simulink model "ntc_measure"  (R2024a)
settings: Solver=ode1be  StartTime=0.0  StopTime=simlength  FixedStep=tc  RelTol=1e-3
undefined symbols (not defined in the file or in its folder): open_loop_gain_opa350, Rntc, tc
libraries: fl_lib x177, ee_lib x28, nesl_utility x26
(part 2 of 2)

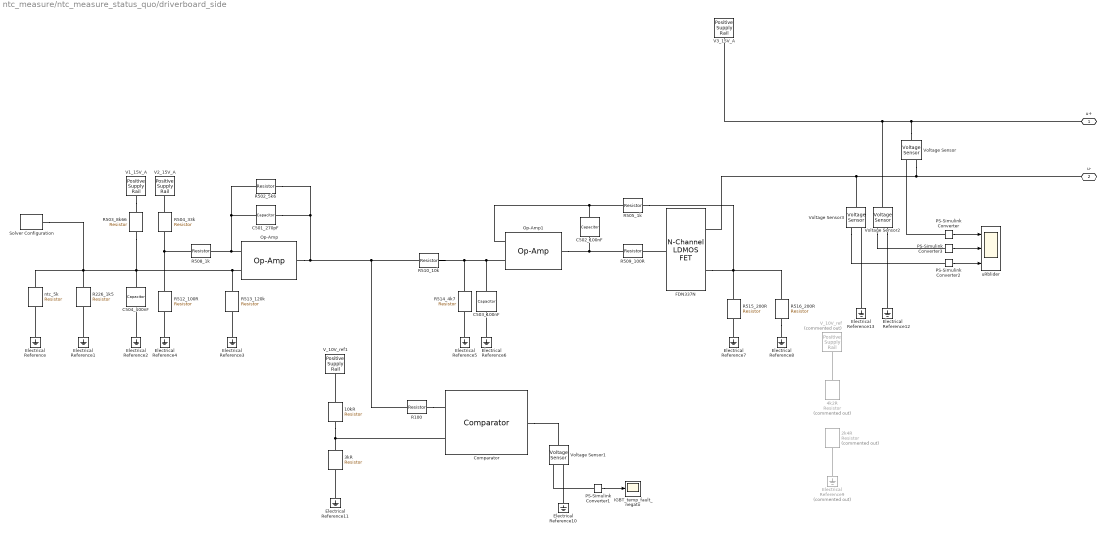
== system ntc_measure/ntc_measure_status_quo/driverboard_side ==
  10kR : fl_lib/Electrical/Electrical Elements/Resistor  R=10e3 Ohm  i_specify=off  i_priority=None  i=0 A  i_nominal_specify=off  i_nominal_value=1  i_nominal_unit=A  v_specify=off  v_priority=None  v=0 V  v_nominal_specify=off  v_nominal_value=1  v_nominal_unit=V
  2k4R : fl_lib/Electrical/Electrical Elements/Resistor  Commented=on  R=2.4e3 Ohm  i_specify=off  i_priority=None  i=0 A  i_nominal_specify=off  i_nominal_value=1  i_nominal_unit=A  v_specify=off  v_priority=None  v=0 V  v_nominal_specify=off  v_nominal_value=1  v_nominal_unit=V
  3kR : fl_lib/Electrical/Electrical Elements/Resistor  R=3e3 Ohm  i_specify=off  i_priority=None  i=0 A  i_nominal_specify=off  i_nominal_value=1  i_nominal_unit=A  v_specify=off  v_priority=None  v=0 V  v_nominal_specify=off  v_nominal_value=1  v_nominal_unit=V
  4k2R : fl_lib/Electrical/Electrical Elements/Resistor  Commented=on  R=4.2e3 Ohm  i_specify=off  i_priority=None  i=0 A  i_nominal_specify=off  i_nominal_value=1  i_nominal_unit=A  v_specify=off  v_priority=None  v=0 V  v_nominal_specify=off  v_nominal_value=1  v_nominal_unit=V
  C501_270pF : fl_lib/Electrical/Electrical Elements/Capacitor  c=270e-12 F  r=1e-6 Ohm  g=0 1/Ohm  i_specify=off  i_priority=None  i=0 A  i_nominal_specify=off  i_nominal_value=1  i_nominal_unit=A  v_specify=off  v_priority=None  v=0 V  v_nominal_specify=off  v_nominal_value=1  v_nominal_unit=V  vc_specify=off  vc_priority=High  vc=0 V  vc_nominal_specify=off  vc_nominal_value=1  vc_nominal_unit=V
  C502_100nF : fl_lib/Electrical/Electrical Elements/Capacitor  c=100e-9 F  r=1e-6 Ohm  g=0 1/Ohm  i_specify=off  i_priority=None  i=0 A  i_nominal_specify=off  i_nominal_value=1  i_nominal_unit=A  v_specify=off  v_priority=None  v=0 V  v_nominal_specify=off  v_nominal_value=1  v_nominal_unit=V  vc_specify=off  vc_priority=High  vc=0 V  vc_nominal_specify=off  vc_nominal_value=1  vc_nominal_unit=V
  C503_100nF : fl_lib/Electrical/Electrical Elements/Capacitor  c=100e-9 F  r=1e-6 Ohm  g=0 1/Ohm  i_specify=off  i_priority=None  i=0 A  i_nominal_specify=off  i_nominal_value=1  i_nominal_unit=A  v_specify=off  v_priority=None  v=0 V  v_nominal_specify=off  v_nominal_value=1  v_nominal_unit=V  vc_specify=off  vc_priority=High  vc=0 V  vc_nominal_specify=off  vc_nominal_value=1  vc_nominal_unit=V
  C504_100nF : fl_lib/Electrical/Electrical Elements/Capacitor  c=100e-9 F  r=1e-6 Ohm  g=0 1/Ohm  i_specify=off  i_priority=None  i=0 A  i_nominal_specify=off  i_nominal_value=1  i_nominal_unit=A  v_specify=off  v_priority=None  v=0 V  v_nominal_specify=off  v_nominal_value=1  v_nominal_unit=V  vc_specify=off  vc_priority=High  vc=0 V  vc_nominal_specify=off  vc_nominal_value=1  vc_nominal_unit=V
  Comparator : ee_lib/Integrated Circuits/Comparator  V_OS=5 mV  C_IN=0 pF  V_OL=0 V  V_OH=5 V  R_OUT=50 Ohm  Delay=0 s
      settings: InternalSimscapePortConfiguration="{\"Bottom\":[],\"Left\":[{\"id\":\"p\",\"label\":\"+\",\"type\":\"foundation.electrical.electrical\"},{\"id\":\"n\",\"label\":\"-\",\"type\":\"foundation.electrical.electrical\"}],\"Right\":[{\"id\":\"J\",\"label\":\"\",\"type\":\"foundation.electrical.electrical\"}],\"Top\":[]}"
  Electrical Reference{,1..8,10..13} (13 alike) : fl_lib/Electrical/Electrical Elements/Electrical Reference
  Electrical Reference9 : fl_lib/Electrical/Electrical Elements/Electrical Reference  Commented=on
  FDN337N : ee_lib/Semiconductors & Converters/N-Channel LDMOS FET  betaref=[11.6, .01] A/V^2  Vfbref=[-1.05, -.1] V  gamma=[3.4, 2.5] V^(1/2)  phib2ref=[.95, .95] V  thesatref=[0, .1] 1/V  theaccdr=0 1/V  alpha=0  Vp=5e-2 V  m=8  Tmeas=25 degC  Rsref=1e-4 Ohm  Rdref=0.07 Ohm  Rgref=8.4 Ohm  Rdriftref=0.1 Ohm  lambda=0.2  Cox=[1600, 1000] pF  Cgso=15 pF  Cgdo=15 pF  Isref=1e-13 A  Vbi=0.6 V  n=1  Cj0=1800 pF  TT=50e-9 s  Tprm=1  Tsim=25 degC  etabet=[1.3, 1.3]  Stvfb=[.0005, .0005] V/K  Stphib=-8.5e-4 V/K  etasat=[1.04, 1.04]  etar=0.95  etardr=0.95  etais=3  Ig_specify=off  Ig_priority=None  Ig=0 A  Ig_nominal_specify=off  Ig_nominal_value=1  Ig_nominal_unit=A  Id_specify=off  Id_priority=None  Id=0 A  Id_nominal_specify=off  Id_nominal_value=1  Id_nominal_unit=A  V_gs_specify=off  V_gs_priority=None  V_gs=0 V  V_gs_nominal_specify=off  V_gs_nominal_value=1  V_gs_nominal_unit=V  V_ds_specify=off  V_ds_priority=None  V_ds=0 V  V_ds_nominal_specify=off  V_ds_nominal_value=1  V_ds_nominal_unit=V  QGoverCox_specify=off  QGoverCox_priority=Low  QGoverCox=0 V  QGoverCox_nominal_specify=off  QGoverCox_nominal_value=1  QGoverCox_nominal_unit=V  QDoverCox_specify=off  QDoverCox_priority=Low  QDoverCox=0 V  QDoverCox_nominal_specify=off  QDoverCox_nominal_value=1  QDoverCox_nominal_unit=V  thermal_network_parameterization=ee.enum.thermalNetworkTopology.junctionCase  Rth=[0, 10] K/W  Rth_Cauer=[1, 3, 10] K/W  Rth_Foster=[4, 6] K/W  thermal_mass_parameterization=ee.enum.thermalNetwork.timeconstant  thermal_mass=[0, 1] J/K  thermal_mass_Cauer=[.1, .3, 1] J/K  thermal_mass_Foster=[1.5, 3] J/K  thermal_time_constant=[0, 10] s  thermal_time_constant_Cauer=[1, 3, 10] s  thermal_time_constant_Foster=[6, 18] s  T0=[25, 25] degC  T0_Cauer=[25, 25, 25] degC  Tvec_initial_Foster=[25, 25, 25, 25] degC
      settings: InternalSimscapePortConfiguration="{\"Bottom\":[],\"Left\":[{\"id\":\"G\",\"label\":\"\",\"type\":\"foundation.electrical.electrical\"}],\"Right\":[{\"id\":\"D\",\"label\":\"d\",\"type\":\"foundation.electrical.electrical\"},{\"id\":\"S\",\"label\":\"s\",\"type\":\"foundation.electrical.electrical\"}],\"Top\":[]}"
  IGBT_temp_fault_negato : Scope
  Op-Amp : fl_lib/Electrical/Electrical Elements/Op-Amp  outI_specify=off  outI_priority=None  outI=0 A  outI_nominal_specify=off  outI_nominal_value=1  outI_nominal_unit=A
  Op-Amp1 : fl_lib/Electrical/Electrical Elements/Op-Amp  outI_specify=off  outI_priority=None  outI=0 A  outI_nominal_specify=off  outI_nominal_value=1  outI_nominal_unit=A
  PS-Simulink Converter{,1..3} (4 alike) : nesl_utility/PS-Simulink Converter  PhysicalDomain=network_engine_domain  SubClassName=ps_output  LeftPortType=input  RightPortType=output  PseudoPeriodic=off  Frequencies=[]  VectorFormat=1-D array  Unit=V  AffineConversion=off
  R100 : fl_lib/Electrical/Electrical Elements/Resistor  R=100 Ohm  i_specify=off  i_priority=None  i=0 A  i_nominal_specify=off  i_nominal_value=1  i_nominal_unit=A  v_specify=off  v_priority=None  v=0 V  v_nominal_specify=off  v_nominal_value=1  v_nominal_unit=V
  R226_1k5 : fl_lib/Electrical/Electrical Elements/Resistor  R=1.5e3 Ohm  i_specify=off  i_priority=None  i=0 A  i_nominal_specify=off  i_nominal_value=1  i_nominal_unit=A  v_specify=off  v_priority=None  v=0 V  v_nominal_specify=off  v_nominal_value=1  v_nominal_unit=V
  R502_5k6 : fl_lib/Electrical/Electrical Elements/Resistor  R=5.6e3 Ohm  i_specify=off  i_priority=None  i=0 A  i_nominal_specify=off  i_nominal_value=1  i_nominal_unit=A  v_specify=off  v_priority=None  v=0 V  v_nominal_specify=off  v_nominal_value=1  v_nominal_unit=V
  R503_8k66 : fl_lib/Electrical/Electrical Elements/Resistor  R=8.66e3 Ohm  i_specify=off  i_priority=None  i=0 A  i_nominal_specify=off  i_nominal_value=1  i_nominal_unit=A  v_specify=off  v_priority=None  v=0 V  v_nominal_specify=off  v_nominal_value=1  v_nominal_unit=V
  R504_33k : fl_lib/Electrical/Electrical Elements/Resistor  R=33e3 Ohm  i_specify=off  i_priority=None  i=0 A  i_nominal_specify=off  i_nominal_value=1  i_nominal_unit=A  v_specify=off  v_priority=None  v=0 V  v_nominal_specify=off  v_nominal_value=1  v_nominal_unit=V
  R505_1k : fl_lib/Electrical/Electrical Elements/Resistor  R=1e3 Ohm  i_specify=off  i_priority=None  i=0 A  i_nominal_specify=off  i_nominal_value=1  i_nominal_unit=A  v_specify=off  v_priority=None  v=0 V  v_nominal_specify=off  v_nominal_value=1  v_nominal_unit=V
  R508_1k : fl_lib/Electrical/Electrical Elements/Resistor  R=1e3 Ohm  i_specify=off  i_priority=None  i=0 A  i_nominal_specify=off  i_nominal_value=1  i_nominal_unit=A  v_specify=off  v_priority=None  v=0 V  v_nominal_specify=off  v_nominal_value=1  v_nominal_unit=V
  R509_100R : fl_lib/Electrical/Electrical Elements/Resistor  R=100 Ohm  i_specify=off  i_priority=None  i=0 A  i_nominal_specify=off  i_nominal_value=1  i_nominal_unit=A  v_specify=off  v_priority=None  v=0 V  v_nominal_specify=off  v_nominal_value=1  v_nominal_unit=V
  R510_10k : fl_lib/Electrical/Electrical Elements/Resistor  R=10e3 Ohm  i_specify=off  i_priority=None  i=0 A  i_nominal_specify=off  i_nominal_value=1  i_nominal_unit=A  v_specify=off  v_priority=None  v=0 V  v_nominal_specify=off  v_nominal_value=1  v_nominal_unit=V
  R512_100R : fl_lib/Electrical/Electrical Elements/Resistor  R=100 Ohm  i_specify=off  i_priority=None  i=0 A  i_nominal_specify=off  i_nominal_value=1  i_nominal_unit=A  v_specify=off  v_priority=None  v=0 V  v_nominal_specify=off  v_nominal_value=1  v_nominal_unit=V
  R513_120k : fl_lib/Electrical/Electrical Elements/Resistor  R=120e3 Ohm  i_specify=off  i_priority=None  i=0 A  i_nominal_specify=off  i_nominal_value=1  i_nominal_unit=A  v_specify=off  v_priority=None  v=0 V  v_nominal_specify=off  v_nominal_value=1  v_nominal_unit=V
  R514_4k7 : fl_lib/Electrical/Electrical Elements/Resistor  R=4.7e3 Ohm  i_specify=off  i_priority=None  i=0 A  i_nominal_specify=off  i_nominal_value=1  i_nominal_unit=A  v_specify=off  v_priority=None  v=0 V  v_nominal_specify=off  v_nominal_value=1  v_nominal_unit=V
  R515_200R : fl_lib/Electrical/Electrical Elements/Resistor  R=200 Ohm  i_specify=off  i_priority=None  i=0 A  i_nominal_specify=off  i_nominal_value=1  i_nominal_unit=A  v_specify=off  v_priority=None  v=0 V  v_nominal_specify=off  v_nominal_value=1  v_nominal_unit=V
  R516_200R : fl_lib/Electrical/Electrical Elements/Resistor  R=200 Ohm  i_specify=off  i_priority=None  i=0 A  i_nominal_specify=off  i_nominal_value=1  i_nominal_unit=A  v_specify=off  v_priority=None  v=0 V  v_nominal_specify=off  v_nominal_value=1  v_nominal_unit=V
  Solver Configuration : nesl_utility/Solver Configuration  PhysicalDomain=network_engine_domain  SubClassName=solver  LeftPortType=input  RightPortType=generic  Tones=[]  Harmonics=[]  SimulateNoise=off  Profile=off  UseLocalSampling=off  EnableSwitchedLinearOptims=on  FrequencyDomain=off  UseCCode=off  RelTol=0.001  AbsTol=0.001  MinStep=1e-09  ToWorkspace=off  RevertToSquareIcSolve=off  NumHomotopyIterations=100  PhasorMode=off  PhasorModeNumHarmonics=1  ConsistencySolver=NEWTON_XTOL_AFTER_FTOL  IndexReductionMethod=DerivativeReplacement  DoDC=off  ResidualTolerance=1e-09  ConsistencyTolSource=GLOBAL  ConsistencyAbsTol=0.001  ConsistencyRelTol=0.001  ConsistencyTolFactor=0.001  UseLocalSolver=on  LocalSolverChoice=NE_BACKWARD_EULER_ADVANCER  ResolveIndetEquations=on  FunctionEvalNumThread=1  LocalSolverSampleTime=tc  DoFixedCost=on  MaxNonlinIter=3  MaxModeIter=2  ComputeImpulses=off  ImpulseIterations=2  LinearAlgebra=auto  LinearAlgebraNumThread=0  EquationFormulation=NE_TIME_EF  DelaysMemoryBudget=1024  AutomaticFiltering=on  FilteringTimeConstant=0.001  PartitionStorageMethod=AS_NEEDED  PartitionMemoryBudget=1024  PartitionMethod=ROBUST  MultibodyUseLocalSolver=off  MultibodyLocalSolverChoice=ODE1  MultibodyLocalSolverSampleTime=0.001
  V1_15V_A : ee_lib/Sources/Positive Supply Rail  v0=15 V
      settings: InternalSimscapePortConfiguration="{\"Bottom\":[],\"Left\":[],\"Right\":[{\"id\":\"p\",\"label\":\"\",\"type\":\"foundation.electrical.electrical\"}],\"Top\":[]}"
  V2_15V_A : ee_lib/Sources/Positive Supply Rail  v0=15 V
      settings: InternalSimscapePortConfiguration="{\"Bottom\":[],\"Left\":[],\"Right\":[{\"id\":\"p\",\"label\":\"\",\"type\":\"foundation.electrical.electrical\"}],\"Top\":[]}"
  V3_15V_A : ee_lib/Sources/Positive Supply Rail  v0=15 V
      settings: InternalSimscapePortConfiguration="{\"Bottom\":[],\"Left\":[],\"Right\":[{\"id\":\"p\",\"label\":\"\",\"type\":\"foundation.electrical.electrical\"}],\"Top\":[]}"
  V_10V_ref : ee_lib/Sources/Positive Supply Rail  Commented=on  v0=10 V
      settings: InternalSimscapePortConfiguration="{\"Bottom\":[],\"Left\":[],\"Right\":[{\"id\":\"p\",\"label\":\"\",\"type\":\"foundation.electrical.electrical\"}],\"Top\":[]}"
  V_10V_ref1 : ee_lib/Sources/Positive Supply Rail  v0=10 V
      settings: InternalSimscapePortConfiguration="{\"Bottom\":[],\"Left\":[],\"Right\":[{\"id\":\"p\",\"label\":\"\",\"type\":\"foundation.electrical.electrical\"}],\"Top\":[]}"
  Voltage Sensor{,1..3} (4 alike) : fl_lib/Electrical/Electrical Sensors/Voltage Sensor
  ntc_5k : fl_lib/Electrical/Electrical Elements/Resistor  R=Rntc Ohm  i_specify=off  i_priority=None  i=0 A  i_nominal_specify=off  i_nominal_value=1  i_nominal_unit=A  v_specify=off  v_priority=None  v=0 V  v_nominal_specify=off  v_nominal_value=1  v_nominal_unit=V
  uRblider : Scope  NumInputPorts=3
  u+ : PMIOPort  Side=Right
  u- : PMIOPort  Port=2  Side=Right
  wires:
  PS-Simulink Converter/1 -> uRblider/1
  PS-Simulink Converter1/1 -> IGBT_temp_fault_negato/1
  PS-Simulink Converter2/1 -> uRblider/3
  PS-Simulink Converter3/1 -> uRblider/2
  connections:
  Electrical Reference7/LConn1 -- R515_200R/RConn1
  Voltage Sensor/LConn1 -- u+/RConn1 -- Voltage Sensor2/LConn1 -- V3_15V_A/RConn1
  R508_1k/LConn1 -- R512_100R/LConn1 -- R504_33k/RConn1
  R503_8k66/RConn1 -- R226_1k5/LConn1 -- Solver Configuration/RConn1 -- ntc_5k/LConn1 -- Op-Amp/LConn1 -- R513_120k/LConn1 -- C504_100nF/LConn1
  Electrical Reference5/LConn1 -- R514_4k7/RConn1
  Voltage Sensor/RConn2 -- u-/RConn1 -- Voltage Sensor3/LConn1 -- FDN337N/RConn1
  R504_33k/LConn1 -- V2_15V_A/RConn1
  Op-Amp1/LConn2 -- C502_100nF/LConn1 -- R505_1k/LConn1
  R508_1k/RConn1 -- Op-Amp/LConn2 -- R502_5k6/LConn1 -- C501_270pF/LConn1
  FDN337N/LConn1 -- R509_100R/RConn1
  FDN337N/RConn2 -- R505_1k/RConn1 -- R515_200R/LConn1 -- R516_200R/LConn1
  Op-Amp1/RConn1 -- C502_100nF/RConn1 -- R509_100R/LConn1
  Electrical Reference/LConn1 -- ntc_5k/RConn1
  V1_15V_A/RConn1 -- R503_8k66/LConn1
  Electrical Reference1/LConn1 -- R226_1k5/RConn1
  Electrical Reference2/LConn1 -- C504_100nF/RConn1
  R510_10k/RConn1 -- C503_100nF/LConn1 -- Op-Amp1/LConn1 -- R514_4k7/LConn1
  C501_270pF/RConn1 -- R100/LConn1 -- R510_10k/LConn1 -- Op-Amp/RConn1 -- R502_5k6/RConn1
  Electrical Reference6/LConn1 -- C503_100nF/RConn1
  Electrical Reference3/LConn1 -- R513_120k/RConn1
  Electrical Reference4/LConn1 -- R512_100R/RConn1
  PS-Simulink Converter/LConn1 -- Voltage Sensor/RConn1
  R516_200R/RConn1 -- Electrical Reference8/LConn1
  4k2R/LConn1 -- V_10V_ref/RConn1
  Electrical Reference9/LConn1 -- 2k4R/RConn1
  R100/RConn1 -- Comparator/LConn1
  Comparator/RConn1 -- Voltage Sensor1/LConn1
  PS-Simulink Converter1/LConn1 -- Voltage Sensor1/RConn1
  Electrical Reference10/LConn1 -- Voltage Sensor1/RConn2
  10kR/RConn1 -- Comparator/LConn2 -- 3kR/LConn1
  Electrical Reference11/LConn1 -- 3kR/RConn1
  10kR/LConn1 -- V_10V_ref1/RConn1
  Voltage Sensor2/RConn2 -- Electrical Reference12/LConn1
  Electrical Reference13/LConn1 -- Voltage Sensor3/RConn2
  Voltage Sensor2/RConn1 -- PS-Simulink Converter3/LConn1
  Voltage Sensor3/RConn1 -- PS-Simulink Converter2/LConn1

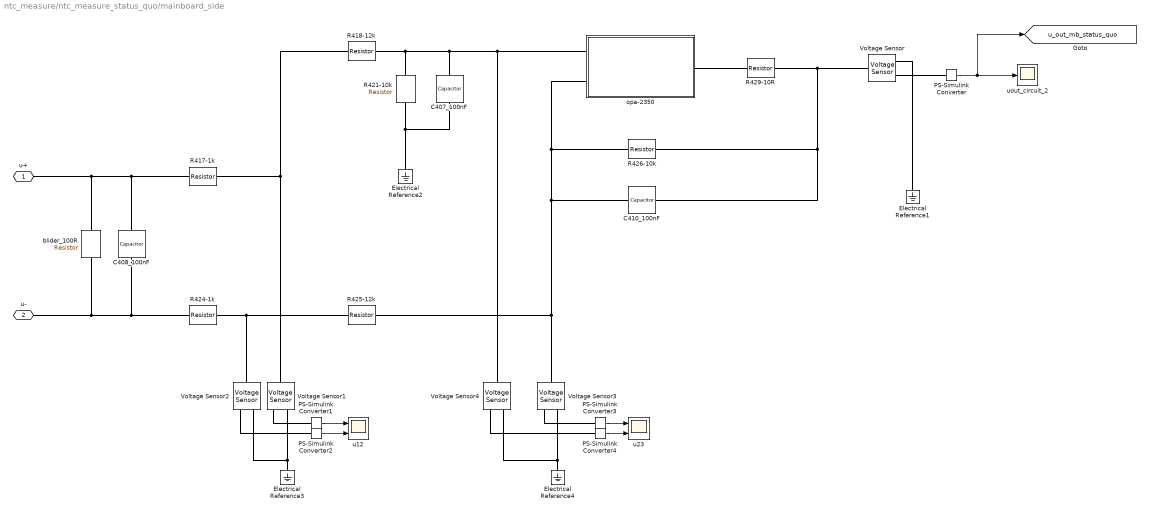
== system ntc_measure/ntc_measure_status_quo/mainboard_side ==
  C407_100nF : fl_lib/Electrical/Electrical Elements/Capacitor  c=100e-9 F  r=1e-6 Ohm  g=0 1/Ohm  i_specify=off  i_priority=None  i=0 A  i_nominal_specify=off  i_nominal_value=1  i_nominal_unit=A  v_specify=off  v_priority=None  v=0 V  v_nominal_specify=off  v_nominal_value=1  v_nominal_unit=V  vc_specify=off  vc_priority=High  vc=0 V  vc_nominal_specify=off  vc_nominal_value=1  vc_nominal_unit=V
  C408_100nF : fl_lib/Electrical/Electrical Elements/Capacitor  c=100e-9 F  r=1e-6 Ohm  g=0 1/Ohm  i_specify=off  i_priority=None  i=0 A  i_nominal_specify=off  i_nominal_value=1  i_nominal_unit=A  v_specify=off  v_priority=None  v=0 V  v_nominal_specify=off  v_nominal_value=1  v_nominal_unit=V  vc_specify=off  vc_priority=High  vc=0 V  vc_nominal_specify=off  vc_nominal_value=1  vc_nominal_unit=V
  C410_100nF : fl_lib/Electrical/Electrical Elements/Capacitor  c=100e-9 F  r=1e-6 Ohm  g=0 1/Ohm  i_specify=off  i_priority=None  i=0 A  i_nominal_specify=off  i_nominal_value=1  i_nominal_unit=A  v_specify=off  v_priority=None  v=0 V  v_nominal_specify=off  v_nominal_value=1  v_nominal_unit=V  vc_specify=off  vc_priority=High  vc=0 V  vc_nominal_specify=off  vc_nominal_value=1  vc_nominal_unit=V
  Electrical Reference{1..4} (4 alike) : fl_lib/Electrical/Electrical Elements/Electrical Reference
  PS-Simulink Converter{,1..4} (5 alike) : nesl_utility/PS-Simulink Converter  PhysicalDomain=network_engine_domain  SubClassName=ps_output  LeftPortType=input  RightPortType=output  PseudoPeriodic=off  Frequencies=[]  VectorFormat=1-D array  Unit=V  AffineConversion=off
  R417-1k : fl_lib/Electrical/Electrical Elements/Resistor  R=1e3 Ohm  i_specify=off  i_priority=None  i=0 A  i_nominal_specify=off  i_nominal_value=1  i_nominal_unit=A  v_specify=off  v_priority=None  v=0 V  v_nominal_specify=off  v_nominal_value=1  v_nominal_unit=V
  R418-12k : fl_lib/Electrical/Electrical Elements/Resistor  R=12e3 Ohm  i_specify=off  i_priority=None  i=0 A  i_nominal_specify=off  i_nominal_value=1  i_nominal_unit=A  v_specify=off  v_priority=None  v=0 V  v_nominal_specify=off  v_nominal_value=1  v_nominal_unit=V
  R421-10k : fl_lib/Electrical/Electrical Elements/Resistor  R=10e3 Ohm  i_specify=off  i_priority=None  i=0 A  i_nominal_specify=off  i_nominal_value=1  i_nominal_unit=A  v_specify=off  v_priority=None  v=0 V  v_nominal_specify=off  v_nominal_value=1  v_nominal_unit=V
  R424-1k : fl_lib/Electrical/Electrical Elements/Resistor  R=1e3 Ohm  i_specify=off  i_priority=None  i=0 A  i_nominal_specify=off  i_nominal_value=1  i_nominal_unit=A  v_specify=off  v_priority=None  v=0 V  v_nominal_specify=off  v_nominal_value=1  v_nominal_unit=V
  R425-12k : fl_lib/Electrical/Electrical Elements/Resistor  R=12e3 Ohm  i_specify=off  i_priority=None  i=0 A  i_nominal_specify=off  i_nominal_value=1  i_nominal_unit=A  v_specify=off  v_priority=None  v=0 V  v_nominal_specify=off  v_nominal_value=1  v_nominal_unit=V
  R426-10k : fl_lib/Electrical/Electrical Elements/Resistor  R=10e3 Ohm  i_specify=off  i_priority=None  i=0 A  i_nominal_specify=off  i_nominal_value=1  i_nominal_unit=A  v_specify=off  v_priority=None  v=0 V  v_nominal_specify=off  v_nominal_value=1  v_nominal_unit=V
  R429-10R : fl_lib/Electrical/Electrical Elements/Resistor  R=10 Ohm  i_specify=off  i_priority=None  i=0 A  i_nominal_specify=off  i_nominal_value=1  i_nominal_unit=A  v_specify=off  v_priority=None  v=0 V  v_nominal_specify=off  v_nominal_value=1  v_nominal_unit=V
  Voltage Sensor{,1..4} (5 alike) : fl_lib/Electrical/Electrical Sensors/Voltage Sensor
  blider_100R : fl_lib/Electrical/Electrical Elements/Resistor  R=100 Ohm  i_specify=off  i_priority=None  i=0 A  i_nominal_specify=off  i_nominal_value=1  i_nominal_unit=A  v_specify=off  v_priority=None  v=0 V  v_nominal_specify=off  v_nominal_value=1  v_nominal_unit=V
  opa-2350 : Subsystem  mask{V_opamp_pos=3.6, V_opamp_neg=-1.6, A=open_loop_gain_opa350}
      mask prompts: V_opamp_pos "V+"; V_opamp_neg "V-"; A "Open Loop Gain"
      mask help: rail to rail op-amp
      mask Help: eval('open opa2350.pdf')
      mask Display:
      | disp('OPA-2350');
      | port_label('lconn', 1, 'in(+)');
      | port_label('lconn', 2, 'in(-)');
      | port_label('rconn', 1, 'out');
  u12 : Scope  NumInputPorts=2
  u23 : Scope  NumInputPorts=2
  uout_circuit_2 : Scope
  u+ : PMIOPort  Side=Left
  u- : PMIOPort  Port=2  Side=Left
  tag scope: u_out_mb_status_quo=global
  wires:
  PS-Simulink Converter/1 -> [u_out_mb_status_quo], uout_circuit_2/1
  PS-Simulink Converter1/1 -> u12/1
  PS-Simulink Converter2/1 -> u12/2
  PS-Simulink Converter4/1 -> u23/2
  PS-Simulink Converter3/1 -> u23/1
  connections:
  R429-10R/LConn1 -- opa-2350/RConn1
  opa-2350/LConn2 -- C410_100nF/LConn1 -- R425-12k/LConn1 -- Voltage Sensor3/LConn1 -- R426-10k/LConn1
  u+/RConn1 -- blider_100R/LConn1 -- R417-1k/RConn1 -- C408_100nF/LConn1
  u-/RConn1 -- blider_100R/RConn1 -- R424-1k/RConn1 -- C408_100nF/RConn1
  Voltage Sensor1/LConn1 -- R417-1k/LConn1 -- R418-12k/RConn1
  Voltage Sensor2/LConn1 -- R424-1k/LConn1 -- R425-12k/RConn1
  opa-2350/LConn1 -- Voltage Sensor4/LConn1 -- C407_100nF/LConn1 -- R421-10k/LConn1 -- R418-12k/LConn1
  Electrical Reference2/LConn1 -- C407_100nF/RConn1 -- R421-10k/RConn1
  R429-10R/RConn1 -- C410_100nF/RConn1 -- R426-10k/RConn1 -- Voltage Sensor/LConn1
  Voltage Sensor/RConn2 -- Electrical Reference1/LConn1
  PS-Simulink Converter/LConn1 -- Voltage Sensor/RConn1
  Voltage Sensor1/RConn1 -- PS-Simulink Converter1/LConn1
  Voltage Sensor1/RConn2 -- Voltage Sensor2/RConn2 -- Electrical Reference3/LConn1
  Voltage Sensor2/RConn1 -- PS-Simulink Converter2/LConn1
  Voltage Sensor3/RConn2 -- Electrical Reference4/LConn1 -- Voltage Sensor4/RConn2
  Voltage Sensor4/RConn1 -- PS-Simulink Converter4/LConn1
  Voltage Sensor3/RConn1 -- PS-Simulink Converter3/LConn1

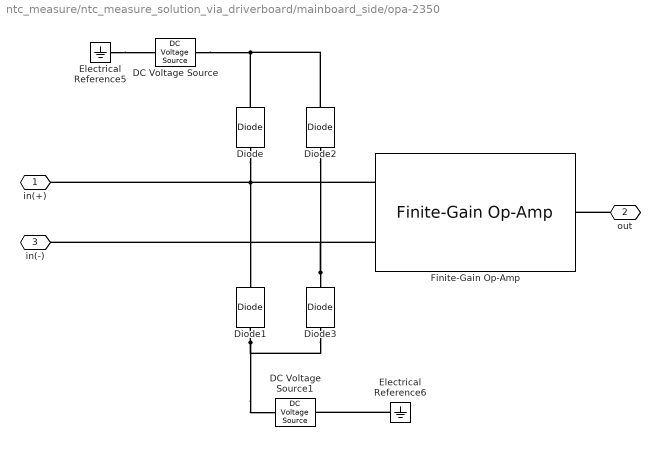
== system ntc_measure/ntc_measure_solution_via_driverboard/mainboard_side/opa-2350 ==
  DC Voltage Source : fl_lib/Electrical/Electrical Sources/DC Voltage Source  v0=V_opamp_pos V
  DC Voltage Source1 : fl_lib/Electrical/Electrical Sources/DC Voltage Source  v0=V_opamp_neg V
  Diode{,1..3} (4 alike) : ee_lib/Semiconductors & Converters/Diode  ModelType=ee.enum.diode.modelType.pwl  TableType=ee.enum.diode.tableType.IfMat  IfMat=[.07, .12, .19, 1.75, 4.24, 7.32, 11.2; .16, .3, .72, 2.14, 5.02, 8.35, 13.12] A  VfMat=[.9, 1.15, 1.25, 1.5, 1.75, 2.17, 2.6, 2.85; .58, .68, .75, 1.1, 1.38, 1.77, 2.27, 2.7] V  TjVec=[25, 125] degC  VfVec=[.5, .7, .9, 1.3, 1.7, 2.1, 2.5] V  IfVec=[.1, .2, .5, 1, 2, 4, 7, 10] A  IrMat=[1e-06, 2e-06, 5e-06, 1e-05, 2.5e-05, 5e-05, .0001; 2e-06, 5e-06, 1e-05, 4e-05, 8e-05, .0002, .0005] A  VrMat=[10, 100, 200, 250, 300, 325, 350; 10, 70, 160, 220, 270, 300, 320] V  VrVec=[10, 20, 40, 50, 70, 80, 100] V  IrVec=[1e-06, 2e-06, 5e-06, 1e-05, 2e-05, 5e-05, .0001] A  Vf=0.6 V  Ron=0.3 Ohm  Goff=1e-8 S  prmExp=ee.enum.diode.expParam.useTwo  I12=[.0137, .545] A  V12=[.6, .7] V  RS=0 Ohm  Tmeas=25 degC  IS=1e-12 A  ec=1  I1=0.0137 A  V1=0.6 V  N_series=1  N_parallel=1  ZenerEnable=false  Rz=0.3 Ohm  BV=inf V  C_param=ee.enum.diode.capParam.fixed  CJ=0 pF  CJ0=5 pF  Vvec=[.1, 10, 100] V  Cvec=[3.5, 1, .4] pF  VJ=1 V  Mgrad=0.5  FC=0.5  Q_param=ee.enum.diode.recoveryParam.off  iRM=-7.15 A  iF=4 A  didt=-750 A/us  trr_factor=3  trr=115 ns  Qrr=150 nA*s  Vr=-600 V  Ls=150 nH  Erec=0.03 J  TT=50 ns  tau=100 ns  T_param=ee.enum.diode.temperatureParam.off  Tdevice=25 degC  I1_T2=0.245 A  V1_T2=0.5 V  IS_T2=1.25e-7 A  Tmeas2=125 degC  XTI_param=ee.enum.diode.xtiParam.pn  XTI=3  EG_param=ee.enum.diode.egapParam.material_si  EG=1.11 eV  dBVdT=0 V/K  enable_faults=simscape.enum.onoff.off  fault_action=simscape.enum.assert.action.none  fault_types=ee.enum.diode.faults.open  tau_fault=1e-3 s  IfMat_faulted=[.07, .12, .19, 1.75, 4.24, 7.32, 11.2; .16, .3, .72, 2.14, 4.02, 6.35, 9.12] A  VfMat_faulted=[.9, 1.15, 1.25, 1.5, 1.75, 2.17, 2.6, 2.85; .58, .68, .75, 1.1, 1.38, 1.77, 2.27, 2.7] V  VfVec_faulted=[.5, .7, .9, 1.3, 1.7, 2.1, 2.5] V  IfVec_faulted=[.1, .2, .5, 1, 2, 4, 7, 10] A  IrMat_faulted=[1e-06, 2e-06, 5e-06, 1e-05, 2.5e-05, 5e-05, .0001; 2e-06, 5e-06, 1e-05, 4e-05, 8e-05, .0002, .0005] A  VrMat_faulted=[1, 10, 20, 25, 30, 32.5, 35; 1, 5, 10, 20, 25, 30, 32] V  VrVec_faulted=[1, 2, 4, 5, 7, 8, 10] V  IrVec_faulted=[1e-06, 2e-06, 5e-06, 1e-05, 2e-05, 5e-05, .0001] A  Ropen_faulted=1000 Ohm  Gshort_faulted=1000 1/Ohm  Vf_faulted=0.6 V  Ron_faulted=0.3 Ohm  Goff_faulted=1e-8 S  I12_faulted=[.0137, .545] A  V12_faulted=[.6, .7] V  IS_faulted=1e-12 A  ec_faulted=1  I1_faulted=0.0137 A  V1_faulted=0.6 V  RS_faulted=0 Ohm  Rz_faulted=0.3 Ohm  BV_faulted=inf V  Cscale_faulted=100  fault_trigger=ee.enum.faults.faultTrigger.temporal  t_fault=inf s  max_permissible_voltage=inf V  n_fail_on_voltage=1  max_permissible_current=inf A  t_fail_on_current=1 s  max_permissible_dVdt=inf V/s  enable_fault_input=simscape.enum.onoff.off  i_specify=off  i_priority=None  i=0 A  i_nominal_specify=off  i_nominal_value=1  i_nominal_unit=A  v_specify=off  v_priority=None  v=0 V  v_nominal_specify=off  v_nominal_value=1  v_nominal_unit=V  v_capacitor_specify=off  v_capacitor_priority=None  v_capacitor=0 V  v_capacitor_nominal_specify=off  v_capacitor_nominal_value=1  v_capacitor_nominal_unit=V  Qj_specify=off  Qj_priority=High  Qj=0 C  Qj_nominal_specify=off  Qj_nominal_value=1  Qj_nominal_unit=C  faulted_specify=off  faulted_priority=None  faulted=0  faulted_nominal_specify=off  faulted_nominal_value=1  faulted_nominal_unit=1  i_diode_specify=off  i_diode_priority=None  i_diode=0 A  i_diode_nominal_specify=off  i_diode_nominal_value=1  i_diode_nominal_unit=A  v_diode_specify=off  v_diode_priority=None  v_diode=0 V  v_diode_nominal_specify=off  v_diode_nominal_value=1  v_diode_nominal_unit=V  i_capacitor_specify=off  i_capacitor_priority=None  i_capacitor=0 A  i_capacitor_nominal_specify=off  i_capacitor_nominal_value=1  i_capacitor_nominal_unit=A  power_dissipated_specify=off  power_dissipated_priority=None  power_dissipated=0 W  power_dissipated_nominal_specify=off  power_dissipated_nominal_value=1  power_dissipated_nominal_unit=W  fidelity_level=ee.enum.diode.fidelity.includeChargeDyn  rec_loss_model=ee.enum.diode.reverseRecoveryModel.fixed  ErecVal=0 J  scaleWithIandV=true  ErecMat=zeros(2, 3) J  TjrecVec=[298.15, 398.15] K  IfrecVec=[.1, 1, 10] A  IrecVal=10 A  VrecVal=10 V  tFilter=1 / 1000 / 100 s  max_permissible_temperature=inf K  t_fail_on_temperature=1 s  thermal_network_parameterization=ee.enum.thermalNetworkTopology.junctionCase  Rth=[0, 10] K/W  Rth_Cauer=[1, 3, 10] K/W  Rth_Foster=[4, 6] K/W  thermal_mass_parameterization=ee.enum.thermalNetwork.timeconstant  thermal_mass=[0, 1] J/K  thermal_mass_Cauer=[.1, .3, 1] J/K  thermal_mass_Foster=[1.5, 3] J/K  thermal_time_constant=[0, 10] s  thermal_time_constant_Cauer=[1, 3, 10] s  thermal_time_constant_Foster=[6, 18] s  thermal_mass_initial_temperatures=[25, 25] degC  thermal_mass_initial_temperatures_Cauer=[25, 25, 25] degC  junction_thermal_mass=0.01 J/K  Tvec_initial_Foster=[25, 25, 25, 25] degC  no_thermal_network=0  junction_temperature_specify=off  junction_temperature_priority=None  junction_temperature=25 degC  junction_temperature_nominal_specify=off  junction_temperature_nominal_value=1  junction_temperature_nominal_unit=degC
  Electrical Reference5 : fl_lib/Electrical/Electrical Elements/Electrical Reference
  Electrical Reference6 : fl_lib/Electrical/Electrical Elements/Electrical Reference
  Finite-Gain Op-Amp : ee_lib/Integrated Circuits/Finite-Gain Op-Amp  A=A  Rin=1e6 Ohm  Rout=100 Ohm  Vmin=V_opamp_neg V  Vmax=V_opamp_pos V  noise_mode=ee.enum.mode.disabled  v_noise=30e-9 V/Hz^(1/2)  noise_prm=ee.enum.ic.noiseParameterization.same  i_noise=0.5e-12 A/Hz^(1/2)  ip_noise=0.5e-12 A/Hz^(1/2)  in_noise=0.5e-12 A/Hz^(1/2)  sample_time=1e-3 s  repeatability=ee.enum.ic.repeatability.notRepeatable  auto_seed_v=1196140742  auto_seed_ip=2348838240  auto_seed_in=4112460543  user_seed_v=0  user_seed_ip=0  user_seed_in=0
      settings: InternalSimscapePortConfiguration="{\"Bottom\":[],\"Left\":[{\"id\":\"p\",\"label\":\"+\",\"type\":\"foundation.electrical.electrical\"},{\"id\":\"n\",\"label\":\"-\",\"type\":\"foundation.electrical.electrical\"}],\"Right\":[{\"id\":\"out\",\"label\":\"\",\"type\":\"foundation.electrical.electrical\"}],\"Top\":[]}"
  in(+) : PMIOPort  Side=Left
  out : PMIOPort  Port=2  Side=Right
  in(-) : PMIOPort  Port=3  Side=Left
  connections:
  Finite-Gain Op-Amp/LConn1 -- in(+)/RConn1 -- Diode1/RConn1 -- Diode/LConn1
  Diode/RConn1 -- DC Voltage Source/LConn1 -- Diode2/RConn1
  out/RConn1 -- Finite-Gain Op-Amp/RConn1
  Diode3/RConn1 -- Diode2/LConn1 -- in(-)/RConn1 -- Finite-Gain Op-Amp/LConn2
  Diode1/LConn1 -- DC Voltage Source1/LConn1 -- Diode3/LConn1
  Electrical Reference6/LConn1 -- DC Voltage Source1/RConn1
  Electrical Reference5/LConn1 -- DC Voltage Source/RConn1

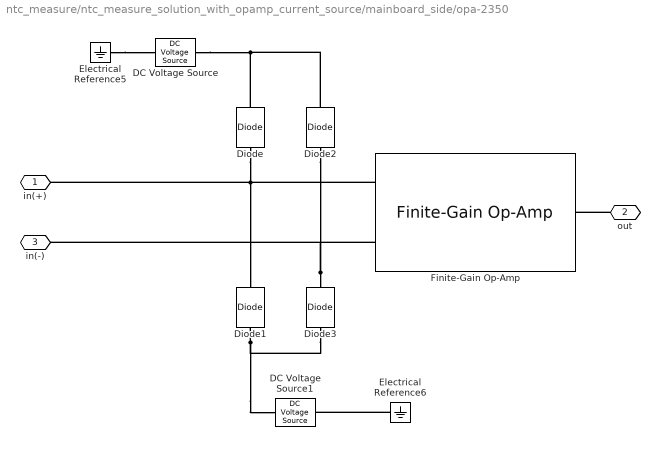
== system ntc_measure/ntc_measure_solution_with_opamp_current_source/mainboard_side/opa-2350 ==
  DC Voltage Source : fl_lib/Electrical/Electrical Sources/DC Voltage Source  v0=V_opamp_pos V
  DC Voltage Source1 : fl_lib/Electrical/Electrical Sources/DC Voltage Source  v0=V_opamp_neg V
  Diode{,1..3} (4 alike) : ee_lib/Semiconductors & Converters/Diode  ModelType=ee.enum.diode.modelType.pwl  TableType=ee.enum.diode.tableType.IfMat  IfMat=[.07, .12, .19, 1.75, 4.24, 7.32, 11.2; .16, .3, .72, 2.14, 5.02, 8.35, 13.12] A  VfMat=[.9, 1.15, 1.25, 1.5, 1.75, 2.17, 2.6, 2.85; .58, .68, .75, 1.1, 1.38, 1.77, 2.27, 2.7] V  TjVec=[25, 125] degC  VfVec=[.5, .7, .9, 1.3, 1.7, 2.1, 2.5] V  IfVec=[.1, .2, .5, 1, 2, 4, 7, 10] A  IrMat=[1e-06, 2e-06, 5e-06, 1e-05, 2.5e-05, 5e-05, .0001; 2e-06, 5e-06, 1e-05, 4e-05, 8e-05, .0002, .0005] A  VrMat=[10, 100, 200, 250, 300, 325, 350; 10, 70, 160, 220, 270, 300, 320] V  VrVec=[10, 20, 40, 50, 70, 80, 100] V  IrVec=[1e-06, 2e-06, 5e-06, 1e-05, 2e-05, 5e-05, .0001] A  Vf=0.6 V  Ron=0.3 Ohm  Goff=1e-8 S  prmExp=ee.enum.diode.expParam.useTwo  I12=[.0137, .545] A  V12=[.6, .7] V  RS=0 Ohm  Tmeas=25 degC  IS=1e-12 A  ec=1  I1=0.0137 A  V1=0.6 V  N_series=1  N_parallel=1  ZenerEnable=false  Rz=0.3 Ohm  BV=inf V  C_param=ee.enum.diode.capParam.fixed  CJ=0 pF  CJ0=5 pF  Vvec=[.1, 10, 100] V  Cvec=[3.5, 1, .4] pF  VJ=1 V  Mgrad=0.5  FC=0.5  Q_param=ee.enum.diode.recoveryParam.off  iRM=-7.15 A  iF=4 A  didt=-750 A/us  trr_factor=3  trr=115 ns  Qrr=150 nA*s  Vr=-600 V  Ls=150 nH  Erec=0.03 J  TT=50 ns  tau=100 ns  T_param=ee.enum.diode.temperatureParam.off  Tdevice=25 degC  I1_T2=0.245 A  V1_T2=0.5 V  IS_T2=1.25e-7 A  Tmeas2=125 degC  XTI_param=ee.enum.diode.xtiParam.pn  XTI=3  EG_param=ee.enum.diode.egapParam.material_si  EG=1.11 eV  dBVdT=0 V/K  enable_faults=simscape.enum.onoff.off  fault_action=simscape.enum.assert.action.none  fault_types=ee.enum.diode.faults.open  tau_fault=1e-3 s  IfMat_faulted=[.07, .12, .19, 1.75, 4.24, 7.32, 11.2; .16, .3, .72, 2.14, 4.02, 6.35, 9.12] A  VfMat_faulted=[.9, 1.15, 1.25, 1.5, 1.75, 2.17, 2.6, 2.85; .58, .68, .75, 1.1, 1.38, 1.77, 2.27, 2.7] V  VfVec_faulted=[.5, .7, .9, 1.3, 1.7, 2.1, 2.5] V  IfVec_faulted=[.1, .2, .5, 1, 2, 4, 7, 10] A  IrMat_faulted=[1e-06, 2e-06, 5e-06, 1e-05, 2.5e-05, 5e-05, .0001; 2e-06, 5e-06, 1e-05, 4e-05, 8e-05, .0002, .0005] A  VrMat_faulted=[1, 10, 20, 25, 30, 32.5, 35; 1, 5, 10, 20, 25, 30, 32] V  VrVec_faulted=[1, 2, 4, 5, 7, 8, 10] V  IrVec_faulted=[1e-06, 2e-06, 5e-06, 1e-05, 2e-05, 5e-05, .0001] A  Ropen_faulted=1000 Ohm  Gshort_faulted=1000 1/Ohm  Vf_faulted=0.6 V  Ron_faulted=0.3 Ohm  Goff_faulted=1e-8 S  I12_faulted=[.0137, .545] A  V12_faulted=[.6, .7] V  IS_faulted=1e-12 A  ec_faulted=1  I1_faulted=0.0137 A  V1_faulted=0.6 V  RS_faulted=0 Ohm  Rz_faulted=0.3 Ohm  BV_faulted=inf V  Cscale_faulted=100  fault_trigger=ee.enum.faults.faultTrigger.temporal  t_fault=inf s  max_permissible_voltage=inf V  n_fail_on_voltage=1  max_permissible_current=inf A  t_fail_on_current=1 s  max_permissible_dVdt=inf V/s  enable_fault_input=simscape.enum.onoff.off  i_specify=off  i_priority=None  i=0 A  i_nominal_specify=off  i_nominal_value=1  i_nominal_unit=A  v_specify=off  v_priority=None  v=0 V  v_nominal_specify=off  v_nominal_value=1  v_nominal_unit=V  v_capacitor_specify=off  v_capacitor_priority=None  v_capacitor=0 V  v_capacitor_nominal_specify=off  v_capacitor_nominal_value=1  v_capacitor_nominal_unit=V  Qj_specify=off  Qj_priority=High  Qj=0 C  Qj_nominal_specify=off  Qj_nominal_value=1  Qj_nominal_unit=C  faulted_specify=off  faulted_priority=None  faulted=0  faulted_nominal_specify=off  faulted_nominal_value=1  faulted_nominal_unit=1  i_diode_specify=off  i_diode_priority=None  i_diode=0 A  i_diode_nominal_specify=off  i_diode_nominal_value=1  i_diode_nominal_unit=A  v_diode_specify=off  v_diode_priority=None  v_diode=0 V  v_diode_nominal_specify=off  v_diode_nominal_value=1  v_diode_nominal_unit=V  i_capacitor_specify=off  i_capacitor_priority=None  i_capacitor=0 A  i_capacitor_nominal_specify=off  i_capacitor_nominal_value=1  i_capacitor_nominal_unit=A  power_dissipated_specify=off  power_dissipated_priority=None  power_dissipated=0 W  power_dissipated_nominal_specify=off  power_dissipated_nominal_value=1  power_dissipated_nominal_unit=W  fidelity_level=ee.enum.diode.fidelity.includeChargeDyn  rec_loss_model=ee.enum.diode.reverseRecoveryModel.fixed  ErecVal=0 J  scaleWithIandV=true  ErecMat=zeros(2, 3) J  TjrecVec=[298.15, 398.15] K  IfrecVec=[.1, 1, 10] A  IrecVal=10 A  VrecVal=10 V  tFilter=1 / 1000 / 100 s  max_permissible_temperature=inf K  t_fail_on_temperature=1 s  thermal_network_parameterization=ee.enum.thermalNetworkTopology.junctionCase  Rth=[0, 10] K/W  Rth_Cauer=[1, 3, 10] K/W  Rth_Foster=[4, 6] K/W  thermal_mass_parameterization=ee.enum.thermalNetwork.timeconstant  thermal_mass=[0, 1] J/K  thermal_mass_Cauer=[.1, .3, 1] J/K  thermal_mass_Foster=[1.5, 3] J/K  thermal_time_constant=[0, 10] s  thermal_time_constant_Cauer=[1, 3, 10] s  thermal_time_constant_Foster=[6, 18] s  thermal_mass_initial_temperatures=[25, 25] degC  thermal_mass_initial_temperatures_Cauer=[25, 25, 25] degC  junction_thermal_mass=0.01 J/K  Tvec_initial_Foster=[25, 25, 25, 25] degC  no_thermal_network=0  junction_temperature_specify=off  junction_temperature_priority=None  junction_temperature=25 degC  junction_temperature_nominal_specify=off  junction_temperature_nominal_value=1  junction_temperature_nominal_unit=degC
  Electrical Reference5 : fl_lib/Electrical/Electrical Elements/Electrical Reference
  Electrical Reference6 : fl_lib/Electrical/Electrical Elements/Electrical Reference
  Finite-Gain Op-Amp : ee_lib/Integrated Circuits/Finite-Gain Op-Amp  A=A  Rin=1e6 Ohm  Rout=100 Ohm  Vmin=V_opamp_neg V  Vmax=V_opamp_pos V  noise_mode=ee.enum.mode.disabled  v_noise=30e-9 V/Hz^(1/2)  noise_prm=ee.enum.ic.noiseParameterization.same  i_noise=0.5e-12 A/Hz^(1/2)  ip_noise=0.5e-12 A/Hz^(1/2)  in_noise=0.5e-12 A/Hz^(1/2)  sample_time=1e-3 s  repeatability=ee.enum.ic.repeatability.notRepeatable  auto_seed_v=3499211588  auto_seed_ip=3890346746  auto_seed_in=545404223  user_seed_v=0  user_seed_ip=0  user_seed_in=0
      settings: InternalSimscapePortConfiguration="{\"Bottom\":[],\"Left\":[{\"id\":\"p\",\"label\":\"+\",\"type\":\"foundation.electrical.electrical\"},{\"id\":\"n\",\"label\":\"-\",\"type\":\"foundation.electrical.electrical\"}],\"Right\":[{\"id\":\"out\",\"label\":\"\",\"type\":\"foundation.electrical.electrical\"}],\"Top\":[]}"
  in(+) : PMIOPort  Side=Left
  out : PMIOPort  Port=2  Side=Right
  in(-) : PMIOPort  Port=3  Side=Left
  connections:
  Finite-Gain Op-Amp/LConn1 -- in(+)/RConn1 -- Diode1/RConn1 -- Diode/LConn1
  Diode/RConn1 -- DC Voltage Source/LConn1 -- Diode2/RConn1
  out/RConn1 -- Finite-Gain Op-Amp/RConn1
  Diode3/RConn1 -- Diode2/LConn1 -- in(-)/RConn1 -- Finite-Gain Op-Amp/LConn2
  Diode1/LConn1 -- DC Voltage Source1/LConn1 -- Diode3/LConn1
  Electrical Reference6/LConn1 -- DC Voltage Source1/RConn1
  Electrical Reference5/LConn1 -- DC Voltage Source/RConn1

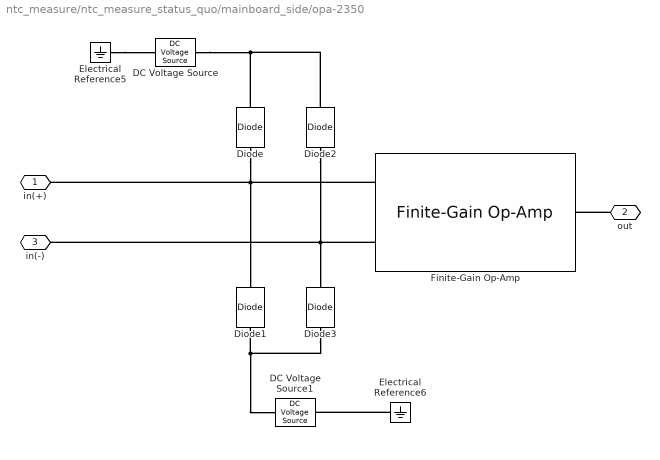
== system ntc_measure/ntc_measure_status_quo/mainboard_side/opa-2350 ==
  DC Voltage Source : fl_lib/Electrical/Electrical Sources/DC Voltage Source  v0=V_opamp_pos V
  DC Voltage Source1 : fl_lib/Electrical/Electrical Sources/DC Voltage Source  v0=V_opamp_neg V
  Diode{,1..3} (4 alike) : ee_lib/Semiconductors & Converters/Diode  ModelType=ee.enum.diode.modelType.pwl  TableType=ee.enum.diode.tableType.IfMat  IfMat=[.07, .12, .19, 1.75, 4.24, 7.32, 11.2; .16, .3, .72, 2.14, 5.02, 8.35, 13.12] A  VfMat=[.9, 1.15, 1.25, 1.5, 1.75, 2.17, 2.6, 2.85; .58, .68, .75, 1.1, 1.38, 1.77, 2.27, 2.7] V  TjVec=[25, 125] degC  VfVec=[.5, .7, .9, 1.3, 1.7, 2.1, 2.5] V  IfVec=[.1, .2, .5, 1, 2, 4, 7, 10] A  IrMat=[1e-06, 2e-06, 5e-06, 1e-05, 2.5e-05, 5e-05, .0001; 2e-06, 5e-06, 1e-05, 4e-05, 8e-05, .0002, .0005] A  VrMat=[10, 100, 200, 250, 300, 325, 350; 10, 70, 160, 220, 270, 300, 320] V  VrVec=[10, 20, 40, 50, 70, 80, 100] V  IrVec=[1e-06, 2e-06, 5e-06, 1e-05, 2e-05, 5e-05, .0001] A  Vf=0.6 V  Ron=0.3 Ohm  Goff=1e-8 S  prmExp=ee.enum.diode.expParam.useTwo  I12=[.0137, .545] A  V12=[.6, .7] V  RS=0 Ohm  Tmeas=25 degC  IS=1e-12 A  ec=1  I1=0.0137 A  V1=0.6 V  N_series=1  N_parallel=1  ZenerEnable=false  Rz=0.3 Ohm  BV=inf V  C_param=ee.enum.diode.capParam.fixed  CJ=0 pF  CJ0=5 pF  Vvec=[.1, 10, 100] V  Cvec=[3.5, 1, .4] pF  VJ=1 V  Mgrad=0.5  FC=0.5  Q_param=ee.enum.diode.recoveryParam.off  iRM=-7.15 A  iF=4 A  didt=-750 A/us  trr_factor=3  trr=115 ns  Qrr=150 nA*s  Vr=-600 V  Ls=150 nH  Erec=0.03 J  TT=50 ns  tau=100 ns  T_param=ee.enum.diode.temperatureParam.off  Tdevice=25 degC  I1_T2=0.245 A  V1_T2=0.5 V  IS_T2=1.25e-7 A  Tmeas2=125 degC  XTI_param=ee.enum.diode.xtiParam.pn  XTI=3  EG_param=ee.enum.diode.egapParam.material_si  EG=1.11 eV  dBVdT=0 V/K  enable_faults=simscape.enum.onoff.off  fault_action=simscape.enum.assert.action.none  fault_types=ee.enum.diode.faults.open  tau_fault=1e-3 s  IfMat_faulted=[.07, .12, .19, 1.75, 4.24, 7.32, 11.2; .16, .3, .72, 2.14, 4.02, 6.35, 9.12] A  VfMat_faulted=[.9, 1.15, 1.25, 1.5, 1.75, 2.17, 2.6, 2.85; .58, .68, .75, 1.1, 1.38, 1.77, 2.27, 2.7] V  VfVec_faulted=[.5, .7, .9, 1.3, 1.7, 2.1, 2.5] V  IfVec_faulted=[.1, .2, .5, 1, 2, 4, 7, 10] A  IrMat_faulted=[1e-06, 2e-06, 5e-06, 1e-05, 2.5e-05, 5e-05, .0001; 2e-06, 5e-06, 1e-05, 4e-05, 8e-05, .0002, .0005] A  VrMat_faulted=[1, 10, 20, 25, 30, 32.5, 35; 1, 5, 10, 20, 25, 30, 32] V  VrVec_faulted=[1, 2, 4, 5, 7, 8, 10] V  IrVec_faulted=[1e-06, 2e-06, 5e-06, 1e-05, 2e-05, 5e-05, .0001] A  Ropen_faulted=1000 Ohm  Gshort_faulted=1000 1/Ohm  Vf_faulted=0.6 V  Ron_faulted=0.3 Ohm  Goff_faulted=1e-8 S  I12_faulted=[.0137, .545] A  V12_faulted=[.6, .7] V  IS_faulted=1e-12 A  ec_faulted=1  I1_faulted=0.0137 A  V1_faulted=0.6 V  RS_faulted=0 Ohm  Rz_faulted=0.3 Ohm  BV_faulted=inf V  Cscale_faulted=100  fault_trigger=ee.enum.faults.faultTrigger.temporal  t_fault=inf s  max_permissible_voltage=inf V  n_fail_on_voltage=1  max_permissible_current=inf A  t_fail_on_current=1 s  max_permissible_dVdt=inf V/s  enable_fault_input=simscape.enum.onoff.off  i_specify=off  i_priority=None  i=0 A  i_nominal_specify=off  i_nominal_value=1  i_nominal_unit=A  v_specify=off  v_priority=None  v=0 V  v_nominal_specify=off  v_nominal_value=1  v_nominal_unit=V  v_capacitor_specify=off  v_capacitor_priority=None  v_capacitor=0 V  v_capacitor_nominal_specify=off  v_capacitor_nominal_value=1  v_capacitor_nominal_unit=V  Qj_specify=off  Qj_priority=High  Qj=0 C  Qj_nominal_specify=off  Qj_nominal_value=1  Qj_nominal_unit=C  faulted_specify=off  faulted_priority=None  faulted=0  faulted_nominal_specify=off  faulted_nominal_value=1  faulted_nominal_unit=1  i_diode_specify=off  i_diode_priority=None  i_diode=0 A  i_diode_nominal_specify=off  i_diode_nominal_value=1  i_diode_nominal_unit=A  v_diode_specify=off  v_diode_priority=None  v_diode=0 V  v_diode_nominal_specify=off  v_diode_nominal_value=1  v_diode_nominal_unit=V  i_capacitor_specify=off  i_capacitor_priority=None  i_capacitor=0 A  i_capacitor_nominal_specify=off  i_capacitor_nominal_value=1  i_capacitor_nominal_unit=A  power_dissipated_specify=off  power_dissipated_priority=None  power_dissipated=0 W  power_dissipated_nominal_specify=off  power_dissipated_nominal_value=1  power_dissipated_nominal_unit=W  fidelity_level=ee.enum.diode.fidelity.includeChargeDyn  rec_loss_model=ee.enum.diode.reverseRecoveryModel.fixed  ErecVal=0 J  scaleWithIandV=true  ErecMat=zeros(2, 3) J  TjrecVec=[298.15, 398.15] K  IfrecVec=[.1, 1, 10] A  IrecVal=10 A  VrecVal=10 V  tFilter=1 / 1000 / 100 s  max_permissible_temperature=inf K  t_fail_on_temperature=1 s  thermal_network_parameterization=ee.enum.thermalNetworkTopology.junctionCase  Rth=[0, 10] K/W  Rth_Cauer=[1, 3, 10] K/W  Rth_Foster=[4, 6] K/W  thermal_mass_parameterization=ee.enum.thermalNetwork.timeconstant  thermal_mass=[0, 1] J/K  thermal_mass_Cauer=[.1, .3, 1] J/K  thermal_mass_Foster=[1.5, 3] J/K  thermal_time_constant=[0, 10] s  thermal_time_constant_Cauer=[1, 3, 10] s  thermal_time_constant_Foster=[6, 18] s  thermal_mass_initial_temperatures=[25, 25] degC  thermal_mass_initial_temperatures_Cauer=[25, 25, 25] degC  junction_thermal_mass=0.01 J/K  Tvec_initial_Foster=[25, 25, 25, 25] degC  no_thermal_network=0  junction_temperature_specify=off  junction_temperature_priority=None  junction_temperature=25 degC  junction_temperature_nominal_specify=off  junction_temperature_nominal_value=1  junction_temperature_nominal_unit=degC
  Electrical Reference5 : fl_lib/Electrical/Electrical Elements/Electrical Reference
  Electrical Reference6 : fl_lib/Electrical/Electrical Elements/Electrical Reference
  Finite-Gain Op-Amp : ee_lib/Integrated Circuits/Finite-Gain Op-Amp  A=A  Rin=1e6 Ohm  Rout=100 Ohm  Vmin=V_opamp_neg V  Vmax=V_opamp_pos V  noise_mode=ee.enum.mode.disabled  v_noise=30e-9 V/Hz^(1/2)  noise_prm=ee.enum.ic.noiseParameterization.same  i_noise=0.5e-12 A/Hz^(1/2)  ip_noise=0.5e-12 A/Hz^(1/2)  in_noise=0.5e-12 A/Hz^(1/2)  sample_time=1e-3 s  repeatability=ee.enum.ic.repeatability.notRepeatable  auto_seed_v=3499211588  auto_seed_ip=3890346746  auto_seed_in=545404223  user_seed_v=0  user_seed_ip=0  user_seed_in=0
      settings: InternalSimscapePortConfiguration="{\"Bottom\":[],\"Left\":[{\"id\":\"p\",\"label\":\"+\",\"type\":\"foundation.electrical.electrical\"},{\"id\":\"n\",\"label\":\"-\",\"type\":\"foundation.electrical.electrical\"}],\"Right\":[{\"id\":\"out\",\"label\":\"\",\"type\":\"foundation.electrical.electrical\"}],\"Top\":[]}"
  in(+) : PMIOPort  Side=Left
  out : PMIOPort  Port=2  Side=Right
  in(-) : PMIOPort  Port=3  Side=Left
  connections:
  Electrical Reference5/LConn1 -- DC Voltage Source/RConn1
  Electrical Reference6/LConn1 -- DC Voltage Source1/RConn1
  Diode3/LConn1 -- DC Voltage Source1/LConn1 -- Diode1/LConn1
  Finite-Gain Op-Amp/LConn2 -- in(-)/RConn1 -- Diode2/LConn1 -- Diode3/RConn1
  out/RConn1 -- Finite-Gain Op-Amp/RConn1
  Diode2/RConn1 -- DC Voltage Source/LConn1 -- Diode/RConn1
  Diode/LConn1 -- Diode1/RConn1 -- in(+)/RConn1 -- Finite-Gain Op-Amp/LConn1
